simulink model "W09_Margin_Check"  (R2024b)
settings: Solver=ode45  StartTime=0.0  StopTime=t_end  MaxStep=0.02  RelTol=1e-3
PreLoadFcn:
  | % W09_Margin_Check 기본 파라미터 (모델을 열 때 자동 실행)
  | % 기본 플랜트는 강의자료 6장의 예 G = 1 over s(s+1)^2
  | defs = { 'K',0.5 ; 'r_amp',1 ; 'tau_d',0 ; 't_end',60 ;
  |          'numG',1 ; 'denG',[1 2 1 0] };
  | for ii = 1:size(defs,1)
  |     if ~evalin('base', sprintf('exist(''%s'',''var'')', defs{ii,1}))
  |         assignin('base', defs{ii,1}, defs{ii,2});
  |     end
  | end
  | clear defs ii
values from neighbouring files (symbols this model uses):
  K = 0.5    [W09_02_pm_to_time.m]    (also in W09_03_run_simulink.m; W09_07_examples.m)
  r_amp = 1    [W09_03_run_simulink.m]
  tau_d = tau_list(i)    [W09_03_run_simulink.m]    (also in W09_07_examples.m)
undefined symbols (not defined in the file or in its folder): denG, numG
settings Model: Creator=admin  LastModifiedBy=admin

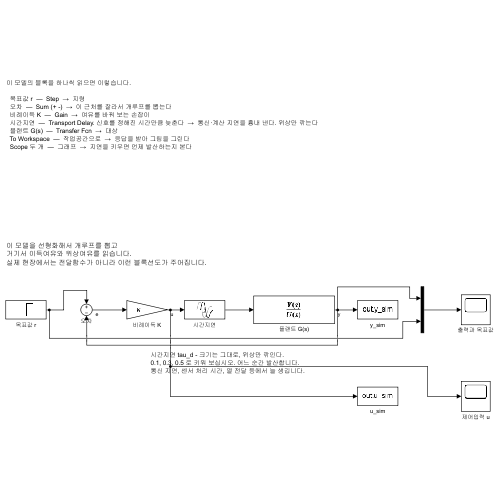
[thumbnail: Simulink's stored preview of the top-level diagram]
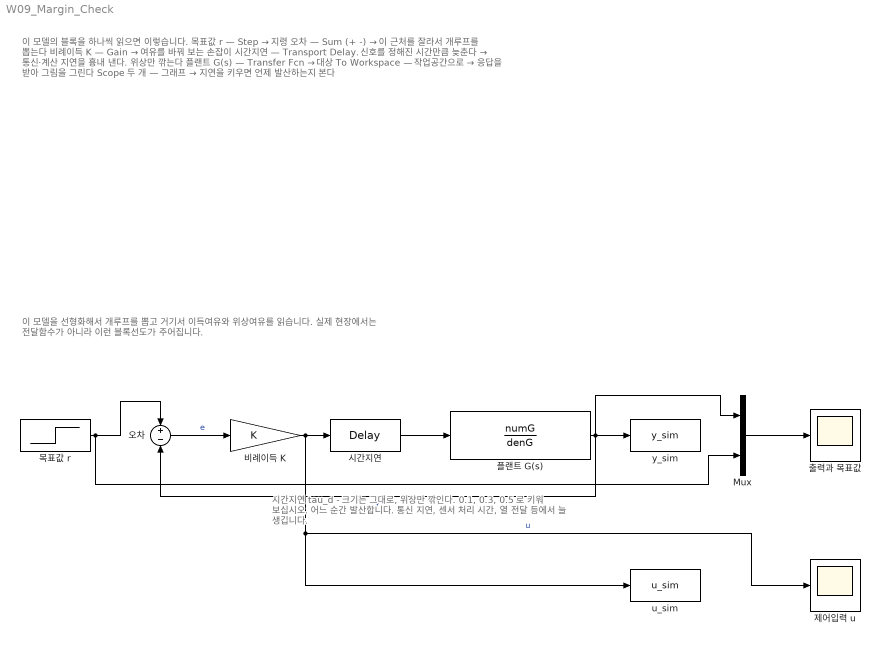
== system W09_Margin_Check ==
  note: 이 모델을 선형화해서 개루프를 뽑고
      | 거기서 이득여유와 위상여유를 읽습니다.
      | 실제 현장에서는 전달함수가 아니라 이런 블록선도가 주어집니다.
  note: 시간지연 tau_d - 크기는 그대로, 위상만 깎인다.
      | 0.1, 0.3, 0.5 로 키워 보십시오. 어느 순간 발산합니다.
      | 통신 지연, 센서 처리 시간, 열 전달 등에서 늘 생깁니다.
  note: 이 모델의 블록을 하나씩 읽으면 이렇습니다.
      |
      |   목표값 r  —  Step  →  지령
      |   오차  —  Sum (+ -)  →  이 근처를 잘라서 개루프를 뽑는다
      |   비례이득 K  —  Gain  →  여유를 바꿔 보는 손잡이
      |   시간지연  —  Transport Delay. 신호를 정해진 시간만큼 늦춘다  →  통신·계산 지연을 흉내 낸다. 위상만 깎는다
      |   플랜트 G(s)  —  Transfer Fcn  →  대상
      |   To Workspace  —  작업공간으로  →  응답을 받아 그림을 그린다
      |   Scope 두 개  —  그래프  →  지연을 키우면 언제 발산하는지 본다
  Mux : Mux  Inputs=2
  u_sim : ToWorkspace  VariableName=u_sim  SaveFormat=Timeseries  SampleTime=-1
  y_sim : ToWorkspace  VariableName=y_sim  SaveFormat=Timeseries  SampleTime=-1
  목표값 r : Step  Time=0  After=r_amp  SampleTime=0
  비례이득 K : Gain  Gain=K
  시간지연 : TransportDelay  DelayTime=tau_d
  오차 : Sum  Inputs=+-
  제어입력 u : Scope
  출력과 목표값 : Scope
  플랜트 G(s) : TransferFcn  Numerator=numG  Denominator=denG
  wires:
  목표값 r/1 -> 오차/1, Mux/2
  오차/1 -> 비례이득 K/1  "e"
  비례이득 K/1 -> u_sim/1, 제어입력 u/1, 시간지연/1  "u"
  시간지연/1 -> 플랜트 G(s)/1
  플랜트 G(s)/1 -> y_sim/1, 오차/2, Mux/1  "y"
  Mux/1 -> 출력과 목표값/1
